simulink model "Closed_loop_PI_speed_control_of_chopper_fed_DC motor"  (R2024a)
settings: Solver=VariableStepAuto  StartTime=0.0  StopTime=5  RelTol=1e-3
libraries: spsGroundLib x4, spsDCVoltageSourceLib x2, spsDCMachineLib x1, spsDiodeLib x1, spsGtoLib x1, spsSeriesRLCBranchLib x1, spsVoltageMeasurementLib x1, spspowerguiLib x1
settings Model: Creator=haris  LastModifiedBy=haris

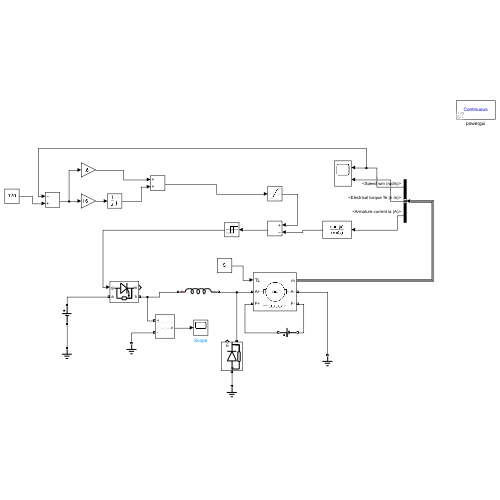
[thumbnail: Simulink's stored preview of the top-level diagram]
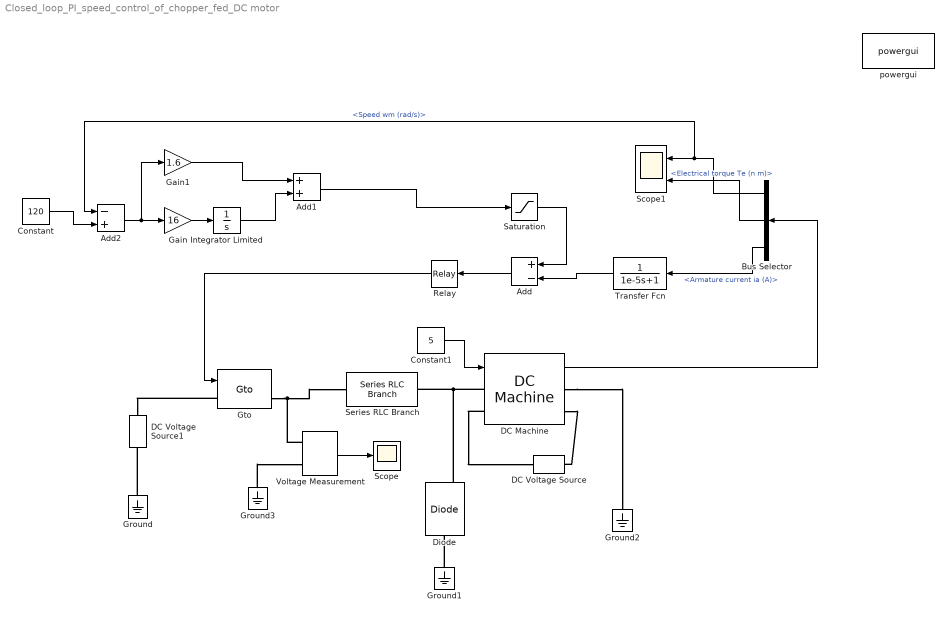
== system Closed_loop_PI_speed_control_of_chopper_fed_DC motor ==
  Add : Sum  Inputs=+-
  Add1 : Sum
  Add2 : Sum  Inputs=-+
  Bus Selector : BusSelector  OutputSignals=Speed wm (rad/s),Electrical torque Te (n m),Armature current ia (A)
  Constant : Constant  Value=120
  Constant1 : Constant  Value=5
  DC Machine : spsDCMachineLib/DC Machine  PresetModel=No  MechanicalLoad=Torque TL  FieldType=Wound  ShowDetailedParameters=on  MeasurementBus=off  RLa="[ 0.6  0.012]"  RLf="[ 240  120]"  Laf=1.8  MachineConstant=Torque constant (N.m/A)  Ke=1.8  Kt=1.8  J=1  Bm=0  Tf=0  w0=1  Ifinit=1.16666666666667  TsPowergui=0  TsBlock=-1
  DC Voltage Source : spsDCVoltageSourceLib/DC Voltage Source  Amplitude=280  Measurements=None
  DC Voltage Source1 : spsDCVoltageSourceLib/DC Voltage Source  Amplitude=240  Measurements=None
  Diode : spsDiodeLib/Diode  Ron=0.001  Lon=0  Vf=0.8  IC=0  UseSnubber=0  Rs=500  Cs=250e-9  Measurements=on
  Gain : Gain  Gain=16
  Gain1 : Gain  Gain=1.6
  Ground{,1..3} (4 alike) : spsGroundLib/Ground  LConnTagsString=a
  Gto : spsGtoLib/Gto  Ron=0.001  Lon=0  Vf=1  Tf=10e-6  Tt=20e-6  IC=0  Rs=1e5  Cs=inf  Measurements=on
      settings: LibrarySourceBlock=sps_lib/Power Electronics/Gto
  Integrator Limited : Integrator  LimitOutput=on  UpperSaturationLimit=+inf
  Relay : Relay
  Saturation : Saturate  UpperLimit=30  LowerLimit=-30
  Scope : Scope
  Scope1 : Scope  NumInputPorts=2
  Series RLC Branch : spsSeriesRLCBranchLib/Series RLC Branch  LConnTagsString=__new0  RConnTagsString=__new0  BranchType=L  Resistance=1  Inductance=1e-3  SetiL0=off  InitialCurrent=0  Capacitance=1e-6  Setx0=off  InitialVoltage=0  Measurements=None
  Transfer Fcn : TransferFcn  Denominator=[1e-5 1]
  Voltage Measurement : spsVoltageMeasurementLib/Voltage Measurement  PhasorSimulation=off  OutputType=Complex  PSBequivalent=0
  powergui : spspowerguiLib/powergui  Priority=1  SimulationMode=Continuous  SampleTime=50e-6  frequency=60  Iterations=50  frequencyindice=0  Pbase=100e6  ErrMax=1e-4  UnitsV=kV  UnitsW=MW  buscounter=0  FunctionMessages=off  echomessages=off  EnableUseOfTLC=off  CurrentSourceSwitches=off  DisableSnubberDevices=off  DisableRonSwitches=off  DisableVfSwitches=off  DisplayEquations=off  AutomaticDiscreteSolvers=off  SolverType=Tustin/Backward Euler (TBE)  Interpol=off  ExternalGateDelay=off  methode=off  Ts=100  x0status=blocks  SPID=on  SwTol=0  HookPort=off  NonlinearTolerance=1e-4  nMaxIteration=100  ContinueOnMaxIteration=off  RestoreLinks=warning  ResistiveCurrentMeasurement=off  Frange=[0:2:500]  Ylog=off  Xlog=on  ShowGrid=off  save=off  variable=ZData  structure=0  ZoomFFT=off  StartTime=0.0  cycles=1  DisplayStyle=1  fundamental=60  FreqAxis=off  MaxFrequency=1000  frequencyindicesteady=1  RmsSteady=1  display=off
  wires:
  Voltage Measurement/1 -> Scope/1
  Constant1/1 -> DC Machine/1
  DC Machine/1 -> Bus Selector/1
  Bus Selector/1 -> Add2/1, Scope1/1  "<Speed wm (rad/s)>"
  Bus Selector/2 -> Scope1/2  "<Electrical torque Te (n m)>"
  Bus Selector/3 -> Transfer Fcn/1  "<Armature current ia (A)>"
  Transfer Fcn/1 -> Add/2
  Add/1 -> Relay/1
  Relay/1 -> Gto/1
  Saturation/1 -> Add/1
  Add1/1 -> Saturation/1
  Gain1/1 -> Add1/1
  Gain/1 -> Integrator Limited/1
  Integrator Limited/1 -> Add1/2
  Add2/1 -> Gain1/1, Gain/1
  Constant/1 -> Add2/2
  connections:
  Gto/LConn1 -- DC Voltage Source1/RConn1
  Ground/LConn1 -- DC Voltage Source1/LConn1
  Gto/RConn1 -- Series RLC Branch/LConn1 -- Voltage Measurement/LConn1
  DC Machine/LConn1 -- Series RLC Branch/RConn1 -- Diode/RConn1
  Ground1/LConn1 -- Diode/LConn1
  DC Machine/LConn2 -- DC Voltage Source/RConn1
  DC Machine/RConn2 -- DC Voltage Source/LConn1
  DC Machine/RConn1 -- Ground2/LConn1
  Ground3/LConn1 -- Voltage Measurement/LConn2
